simulink model "bioreactor_monod_completo"  (R2025b)
settings: Solver=ode15s  StartTime=0.0  StopTime=80  RelTol=1e-6
settings Model: Creator=sergio.castano  LastModifiedBy=Sergio

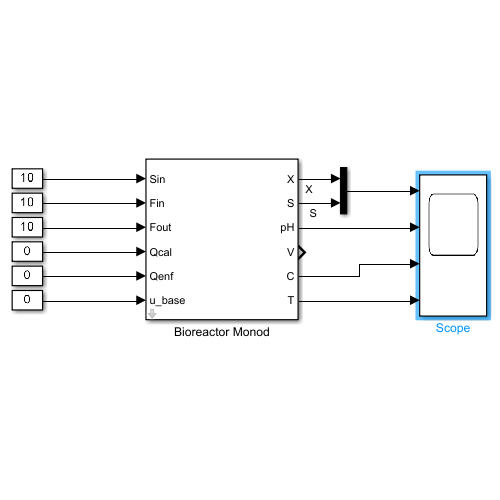
[thumbnail: Simulink's stored preview of the top-level diagram]
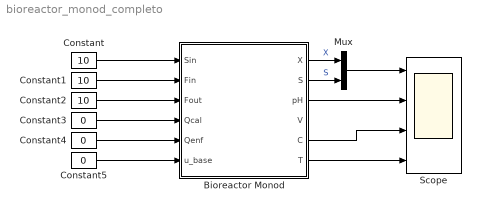
== system bioreactor_monod_completo ==
  Bioreactor Monod : Subsystem  mask(Biorreactor de Monod){Y=0.4, Ks=1.0, umax=0.4, Yxo=0.9, kLa=152.4, Cstar=7.5, YQ=460, rho=1.0, cp=4.18, UA_amb=28.4, Tamb=22, qA=2.0e-3, CT=0.020, pKa=6.8, Kw=1e-14, pH_med=7.0, Ain=0, Xini=0.01, Sini=10, Vini=50, Vmax=75, Cini=7.5, Tini=22, Aini=0}
      mask help:
      | Tanque agitado, seis estados: V, X, S, C, T y A.
      | Unidad de tiempo: la HORA. Caudales en L/h, potencias en kJ/h.
      mask Help:
      | <pre>
      | BIORREACTOR DE MONOD - modelo no lineal de seis estados
      | 
      | ESTADOS
      |    V   [L]       volumen de caldo
      |    X   [g/L]     biomasa
      |    S   [g/L]     sustrato limitante
      |    C   [mg/L]    oxígeno disuelto
      |    T   [°C]      temperatura
      |    A   [mol/L]   ácido neto acumulado, referido al medio fresco
      | 
      | ENTRADAS
      |    Sin      [g/L]         sustrato en la alimentación
      |    Fin      [L/h]         caudal de entrada
      |    Fout     [L/h]         caudal de salida
      |    Qcal     [kJ/h]        potencia de calentamiento
      |    Qenf     [kJ/h]        potencia de enfriamiento
      |    u_base   [mol/(L h)]   dosificación de base
      | 
      | SALIDAS
      |    X, S, pH, V, C, T      el pH se calcula de A, no es un estado
      | 
      | UNIDADES - leer antes de conectar nada
      |    La unidad de tiempo es la HORA, porque umax está en 1/h.
      |    Las potencias térmicas van en kJ/h, NO en vatios:  1 W = 3.6 kJ/h.
      |    C está en mg/L y X en g/L, así que el consumo de oxígeno lleva
      |    el factor 1000 que convierte gramos de biomasa a miligramos de O2.
      | 
      | PARÁMETROS QUE NO APARECEN EN EL DIÁLOGO
      |    Ka y A0 no se escriben: se deducen del tampón y del pH del medio
      |    dentro de los bloques Constant correspondientes.
      | 
      | Curso de Control de Bioprocesos - Universidad EIA
      | </pre>
      mask DialogControl DescGroupVar Prompt: Bioreactor de Monod
      mask DialogControl DescTextVar Prompt: Tanque agitado, seis estados: V, X, S, C, T y A. Unidad de tiempo: la HORA. Caudales en L/h, potencias en kJ/h.
      mask DialogControl Cinetica Prompt: Cinetica
      mask DialogControl Y Tooltip: Y  [gX / gS]   rendimiento biomasa / sustrato
      mask DialogControl Ks Tooltip: Ks  [g / L]   constante de saturacion de Monod
      mask DialogControl umax Tooltip: umax  [1 / h]   velocidad maxima de crecimiento
      mask DialogControl Oxigeno Prompt: Oxigeno y energia
      mask DialogControl Yxo Tooltip: Yxo  [gX / gO2]   rendimiento biomasa / oxigeno
      mask DialogControl kLa Tooltip: kLa  [1 / h]   coeficiente de transferencia
      mask DialogControl Cstar Tooltip: C*  [mg / L]   saturacion de O2 (Henry)
      mask DialogControl YQ Tooltip: YQ  [kJ / mol O2]   calor por mol respirado
      mask DialogControl rho Tooltip: rho  [kg / L]   densidad del caldo
      mask DialogControl cp Tooltip: cp  [kJ / (kg K)]   calor especifico del caldo
      mask DialogControl UA_amb Tooltip: UA  [kJ / (h K)]   perdida al ambiente
      mask DialogControl Tamb Tooltip: Tamb  [C]   temperatura ambiente
      mask DialogControl Acidez Prompt: pH
      mask DialogControl qA Tooltip: qA  [mol / gX]   acido producido por biomasa
      mask DialogControl CT Tooltip: CT  [mol / L]   tampon total del medio
      mask DialogControl pKa Tooltip: pKa  [-]   del tampon
      mask DialogControl Kw Tooltip: Kw  [-]   producto ionico del agua
      mask DialogControl pH_med Tooltip: pH del medio fresco  (define A = 0)
      mask DialogControl Ain Tooltip: Ain  [mol / L]   acido neto en la alimentacion
      mask DialogControl Iniciales Prompt: Iniciales
      mask DialogControl Xini Tooltip: X(0)  [g/L]   inoculo
      mask DialogControl Sini Tooltip: S(0)  [g/L]   sustrato inicial
      mask DialogControl Vini Tooltip: V(0)  [L]   volumen inicial
      mask DialogControl Vmax Tooltip: Vmax  [L]   capacidad del vaso
      mask DialogControl Cini Tooltip: C(0)  [mg / L]   O2 disuelto inicial
      mask DialogControl Tini Tooltip: T(0)  [C]   temperatura inicial
      mask DialogControl Aini Tooltip: A(0)  [mol / L]   acido neto inicial
  Constant : Constant  Value=10
  Constant1 : Constant  Value=10
  Constant2 : Constant  Value=10
  Constant3 : Constant  Value=0
  Constant4 : Constant  Value=0
  Constant5 : Constant  Value=0
  Mux : Mux  Inputs=2
  Scope : Scope  NumInputPorts=4
      settings: ActiveDisplayYMinimum=-1.2387499999999998  ActiveDisplayYMaximum=11.24875
  wires:
  Constant/1 -> Bioreactor Monod/1(Sin)
  Constant1/1 -> Bioreactor Monod/2(Fin)
  Constant2/1 -> Bioreactor Monod/3(Fout)
  Constant3/1 -> Bioreactor Monod/4(Qcal)
  Constant4/1 -> Bioreactor Monod/5(Qenf)
  Constant5/1 -> Bioreactor Monod/6(u_base)
  Bioreactor Monod/3(pH) -> Scope/2
  Bioreactor Monod/2(S) -> Mux/2  "S"
  Bioreactor Monod/1(X) -> Mux/1  "X"
  Mux/1 -> Scope/1
  Bioreactor Monod/5(C) -> Scope/3
  Bioreactor Monod/6(T) -> Scope/4

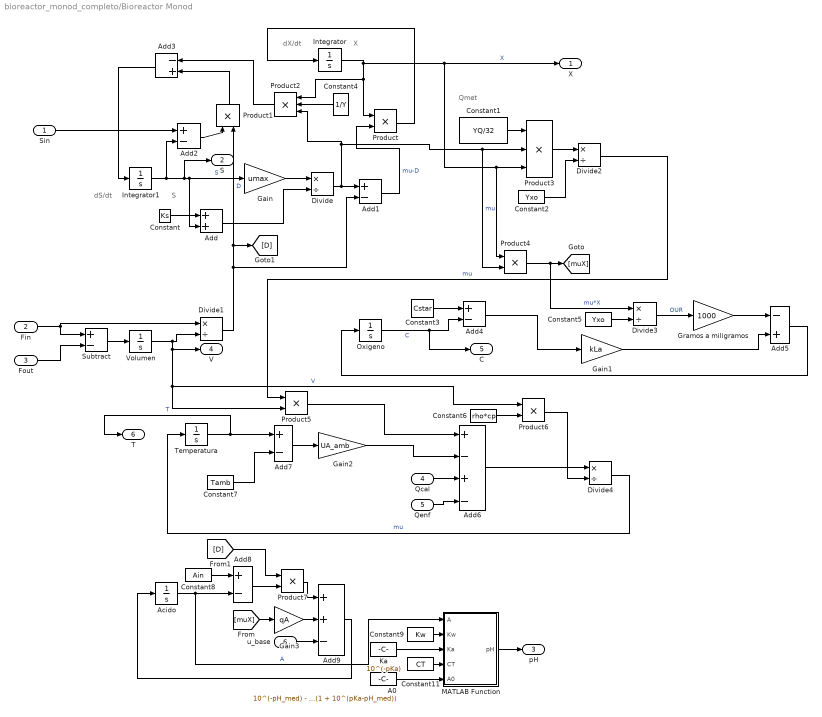
== system bioreactor_monod_completo/Bioreactor Monod ==
  note: Qmet
  note: dX/dt
  note: X
  note: dS/dt
  note: S
  Sin : Inport
  Fin : Inport  Port=2
  Fout : Inport  Port=3
  Qcal : Inport  Port=4
  Qenf : Inport  Port=5
  u_base : Inport  Port=6
  A0 : Constant  Value=10^(-pH_med) - Kw*10^(pH_med) - CT/(1 + 10^(pKa-pH_med))
  Acido : Integrator  InitialCondition=Aini
  Add : Sum
  Add{1..2,4,7..8} (5 alike) : Sum  Inputs=+-
  Add3 : Sum  Inputs=-+
  Add5 : Sum  Inputs=-+
  Add6 : Sum  Inputs=+-+-
  Add9 : Sum  Inputs=++-
  Constant : Constant  Value=Ks
  Constant1 : Constant  Value=YQ/32
  Constant11 : Constant  Value=CT
  Constant2 : Constant  Value=Yxo
  Constant3 : Constant  Value=Cstar
  Constant4 : Constant  Value=1/Y
  Constant5 : Constant  Value=Yxo
  Constant6 : Constant  Value=rho*cp
  Constant7 : Constant  Value=Tamb
  Constant8 : Constant  Value=Ain
  Constant9 : Constant  Value=Kw
  Divide{,1..4} (5 alike) : Product  Inputs=*/
  Gain : Gain  Gain=umax
  Gain1 : Gain  Gain=kLa
  Gain2 : Gain  Gain=UA_amb
  Gain3 : Gain  Gain=qA
  Gramos a miligramos : Gain  Gain=1000
  Integrator : Integrator  InitialCondition=Xini  LimitOutput=on  LowerSaturationLimit=0
  Integrator1 : Integrator  InitialCondition=Sini  LimitOutput=on  LowerSaturationLimit=0
  Ka : Constant  Value=10^(-pKa)
  MATLAB Function : MATLAB Function  TreatAsAtomicUnit=on
  Oxigeno : Integrator  InitialCondition=Cini  LimitOutput=on  LowerSaturationLimit=0
  Product{,1,4..7} (6 alike) : Product
  Product2 : Product  Inputs=3
  Product3 : Product  Inputs=3
  Subtract : Sum  Inputs=+-
  Temperatura : Integrator  InitialCondition=Tini
  Volumen : Integrator  InitialCondition=Vini  LimitOutput=on  UpperSaturationLimit=Vmax  LowerSaturationLimit=0.1
  X : Outport
  S : Outport  Port=2
  pH : Outport  Port=3
  V : Outport  Port=4
  C : Outport  Port=5
  T : Outport  Port=6
  wires:
  Add1/1 -> Product/2  "mu-D"
  Integrator1/1 -> Add2/2, S/1, Add/2, Gain/1  "S"
  Add2/1 -> Product1/1
  Divide1/1 -> Add1/2, [D], Product1/2  "D"
  Product2/1 -> Add3/1
  Integrator/1 -> Product4/1, Product3/3, X/1, Product2/1, Product/1  "X"
  Add3/1 -> Integrator1/1
  Divide/1 -> Product4/2, Product3/2, Product2/3, Add1/1  "mu"
  Add/1 -> Divide/2
  Constant4/1 -> Product2/2
  Sin/1 -> Add2/1
  Constant/1 -> Add/1
  Gain/1 -> Divide/1
  Product/1 -> Integrator/1
  Product1/1 -> Add3/2
  Subtract/1 -> Volumen/1
  Fout/1 -> Subtract/2
  Fin/1 -> Subtract/1, Divide1/1
  Volumen/1 -> Product6/1, Product5/2, V/1, Divide1/2  "V"
  Constant1/1 -> Product3/1
  Product3/1 -> Divide2/1
  Constant2/1 -> Divide2/2
  Constant3/1 -> Add4/1
  Oxigeno/1 -> C/1, Add4/2  "C"
  Add4/1 -> Gain1/1
  Product4/1 -> Divide3/1, [muX]  "mu*X"
  Constant5/1 -> Divide3/2
  Divide3/1 -> Gramos a miligramos/1  "OUR"
  Divide2/1 -> Product5/1  "mu"
  Product5/1 -> Add6/1
  Temperatura/1 -> T/1, Add7/1  "T"
  Constant7/1 -> Add7/2
  Add7/1 -> Gain2/1
  Gain2/1 -> Add6/2
  Qcal/1 -> Add6/3
  Qenf/1 -> Add6/4
  Add6/1 -> Divide4/1
  Constant6/1 -> Product6/2
  Product6/1 -> Divide4/2
  Divide4/1 -> Temperatura/1  "mu"
  Acido/1 -> MATLAB Function/1(A), Add8/2  "A"
  Constant8/1 -> Add8/1
  Gain3/1 -> Add9/2
  [muX] -> Gain3/1
  u_base/1 -> Add9/3
  Add9/1 -> Acido/1
  Constant9/1 -> MATLAB Function/2(Kw)
  Ka/1 -> MATLAB Function/3(Ka)
  Constant11/1 -> MATLAB Function/4(CT)
  A0/1 -> MATLAB Function/5(A0)
  MATLAB Function/1(pH) -> pH/1
  Gramos a miligramos/1 -> Add5/1
  Gain1/1 -> Add5/2
  Add5/1 -> Oxigeno/1
  Add8/1 -> Product7/2
  Product7/1 -> Add9/1
  [D] -> Product7/1

== matlab function bioreactor_monod_completo/Bioreactor Monod/MATLAB Function ==
  data: A input; pH output; Kw input; Ka input; CT input; A0 input
function pH = ph_fcn(A, Kw, Ka, CT, A0)
%PH_FCN  Convierte acido neto acumulado en pH.
%
%  Pegar este codigo DENTRO de un bloque MATLAB Function de Simulink.
%
%  Entradas (A por la senal, el resto como parametros del bloque):
%     A   [mol/L]  acido neto acumulado, referido al medio fresco  (del integrador)
%     Kw  [-]      producto ionico del agua            1e-14
%     Ka  [-]      constante del tampon                10^-6.8
%     CT  [mol/L]  tampon total                        0.020
%     A0  [mol/L]  valor de la funcion de cargas en el pH del medio fresco
%
%  Salida:
%     pH  [-]
%
%  POR QUE HACE FALTA RESOLVER:
%  el balance de cargas da A en funcion de [H+] de forma explicita,
%
%        A = [H+] - Kw/[H+] - CT*Ka/(Ka + [H+])
%
%  pero nosotros necesitamos el camino contrario: dado A, hallar [H+].
%  Esa inversion no tiene formula cerrada (es una cubica), asi que se
%  resuelve numericamente.  Usamos biseccion con un numero FIJO de
%  iteraciones: es lo unico que garantiza que el bloque siempre termina
%  en el mismo tiempo y que el generador de codigo lo acepta.
%
%  La funcion de cargas es MONOTONA DECRECIENTE en pH, lo que hace que la
%  biseccion no pueda fallar: siempre hay una y solo una solucion.

%#codegen

objetivo = A + A0;        % valor absoluto de la funcion de cargas

lo = 0.0;                 % pH minimo del intervalo de busqueda
hi = 14.0;                % pH maximo

for k = 1:40              % 40 iteraciones -> precision ~1e-11 unidades de pH
    mid = 0.5*(lo + hi);
    H   = 10^(-mid);
    f   = H - Kw/H - CT*Ka/(Ka + H);    % funcion de cargas evaluada en mid
    if f > objetivo       % decreciente: si da de mas, el pH real es mayor
        lo = mid;
    else
        hi = mid;
    end
end

pH = 0.5*(lo + hi);
